simulink model "SonModel"  (R2025b)
settings: Solver=ode4  StartTime=0.0  StopTime=30  FixedStep=0.005  RelTol=1e-3
values from neighbouring files (symbols this model uses):
  CA_alpha_rad_vec = [0 2 4 5 6 7 8 9 10 11 12 13 14 15]*pi/180    [CA_RASAero_2DLUT_Gokturk_1stageVson.m]
  CA_Mach_vec = [      0.01 0.02 0.03 0.04 0.05 0.06 0.07 0.08 0.09 0.1 0.11 0.12      0.13 0.14 0.15 0.16 0.17 0.18 0.19 0.2 0.21 0.22 0.23 0.24      0.25 0.26 0.27 0.28 0.29 0.3 0.31 0.32 0.33 0.34 0.35 0.36      0.37 0.38 0.39 0.4 0.41 0.42 0.43 0.44 0.45 0.46 0.47 0.48      0.49 0.5 0.51 0.52 0.53 0.54 0.55 0.56 0.57 0.58 0.59 0.6      0.61 0.62 0.63 0.64 0.65 0.66 0.67 0.68 0.69 0.7 0.71 0.72      0.73 0.74  ...(+14344 chars)    [CA_RASAero_2DLUT_Gokturk_1stageVson.m]
  CA_table = [ ... (first row only)    [CA_RASAero_2DLUT_Gokturk_1stageVson.m]
  CN_alpha_rad_vec = [0 2 4 5 6 7 8 9 10 11 12 13 14 15]*pi/180    [CN_RASAero_2DLUT_Gokturk_1stageVson.m]
  CN_Mach_vec = [      0.01 0.02 0.03 0.04 0.05 0.06 0.07 0.08 0.09 0.1 0.11 0.12      0.13 0.14 0.15 0.16 0.17 0.18 0.19 0.2 0.21 0.22 0.23 0.24      0.25 0.26 0.27 0.28 0.29 0.3 0.31 0.32 0.33 0.34 0.35 0.36      0.37 0.38 0.39 0.4 0.41 0.42 0.43 0.44 0.45 0.46 0.47 0.48      0.49 0.5 0.51 0.52 0.53 0.54 0.55 0.56 0.57 0.58 0.59 0.6      0.61 0.62 0.63 0.64 0.65 0.66 0.67 0.68 0.69 0.7 0.71 0.72      0.73 0.74  ...(+14344 chars)    [CN_RASAero_2DLUT_Gokturk_1stageVson.m]
  CN_table = [ ... (first row only)    [CN_RASAero_2DLUT_Gokturk_1stageVson.m]
  CP_alpha_rad_vec = [0 2 4 5 6 7 8 9 10 11 12 13 14 15]*pi/180    [CP_RASAero_2DLUT_Gokturk_1stageVson.m]
  CP_Mach_vec = [      0.01 0.02 0.03 0.04 0.05 0.06 0.07 0.08 0.09 0.1 0.11 0.12      0.13 0.14 0.15 0.16 0.17 0.18 0.19 0.2 0.21 0.22 0.23 0.24      0.25 0.26 0.27 0.28 0.29 0.3 0.31 0.32 0.33 0.34 0.35 0.36      0.37 0.38 0.39 0.4 0.41 0.42 0.43 0.44 0.45 0.46 0.47 0.48      0.49 0.5 0.51 0.52 0.53 0.54 0.55 0.56 0.57 0.58 0.59 0.6      0.61 0.62 0.63 0.64 0.65 0.66 0.67 0.68 0.69 0.7 0.71 0.72      0.73 0.74  ...(+14344 chars)    [CP_RASAero_2DLUT_Gokturk_1stageVson.m]
  CP_table = [ ... (first row only)    [CP_RASAero_2DLUT_Gokturk_1stageVson.m]
undefined symbols (not defined in the file or in its folder): Cg, dCA_table, dCm_table, dCN_table, delta_max, g, I_total, KTS_alpha_rad_vec, KTS_delta_rad_vec, KTS_Mach_vec, m_propellant, m_rocket, servo_rate, servo_tau, Sref, thrust, time, time2
libraries: simulink_extras x7, simulink x3, aerolibobsolete x1, slpidlib x1, aerolibatmos2 x1
(part 1 of 2)
settings Model: Creator=aliki  LastModifiedBy=aliki

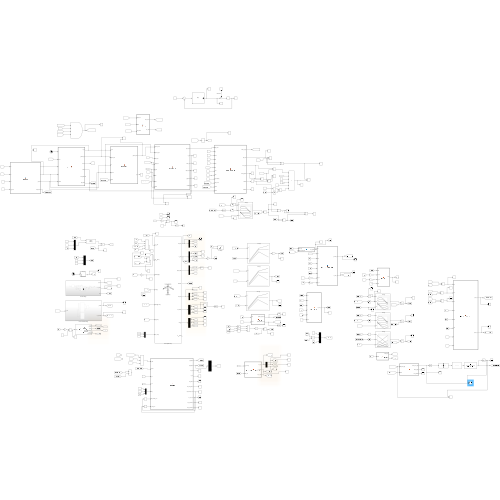
[thumbnail: Simulink's stored preview of the top-level diagram]
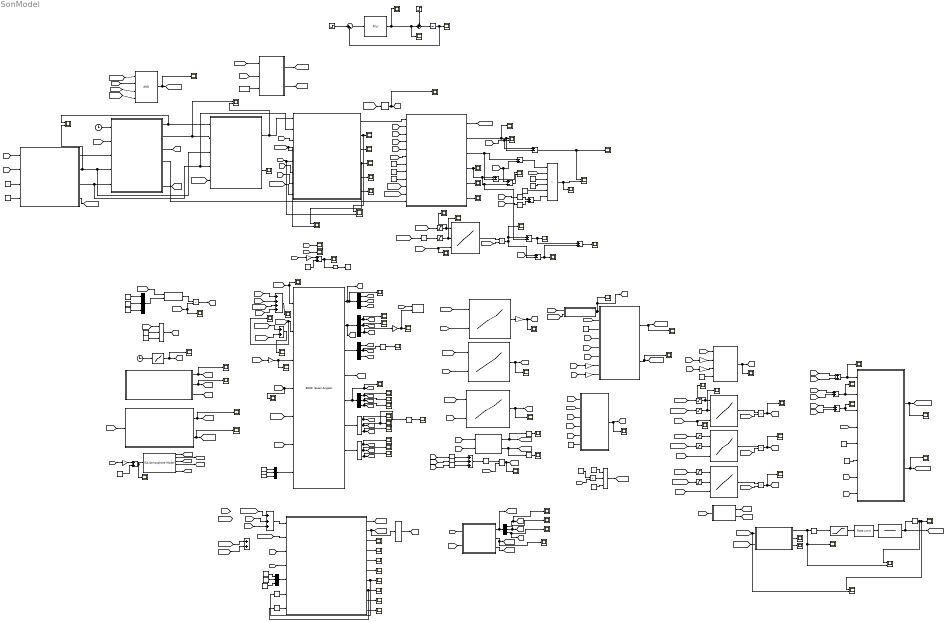
== system SonModel ==
  1-D Lookup Table : Lookup_n-D  NumberOfTableDimensions=1  BreakpointsForDimension1=time2  Table=Cg  InternalRulePriority=Speed  RndMeth=Simplest
  2-D Lookup Table : Lookup_n-D  BreakpointsForDimension1=CA_alpha_rad_vec  BreakpointsForDimension2=CA_Mach_vec  Table=CA_table  ExtrapMethod=Clip  InternalRulePriority=Speed  RndMeth=Simplest
      settings: InputPortMap=u0,u1
  2-D Lookup Table1 : Lookup_n-D  BreakpointsForDimension1=CN_alpha_rad_vec  BreakpointsForDimension2=CN_Mach_vec  Table=CN_table  InternalRulePriority=Speed  RndMeth=Simplest
      settings: InputPortMap=u0,u1
  2-D Lookup Table2 : Lookup_n-D  BreakpointsForDimension1=CP_alpha_rad_vec  BreakpointsForDimension2=CP_Mach_vec  Table=CP_table  InternalRulePriority=Speed  RndMeth=Simplest
      settings: InputPortMap=u0,u1
  6DOF (Quaternion) : aerolibobsolete/6DOF (Euler Angles)  units=Metric (MKS)  mtype=Custom Variable  rep=Quaternion  xme_0=[0 0 0]  Vm_0=[0 0 0]  eul_0=[0 45*pi/180 0]  pm_0=[0 0 0]  mass_0=17.958  mass_e=15.467  mass_f=17.958  inertia=eye(3)  inertia_e=[0.03 0 0; 0 2.263 0; 0 0 2.263]  inertia_f=[0.033 0 0; 0 2.95 0; 0 0 2.95]  k_quat=1.0  vre_flag=on  abi_flag=off  aMode=0  xme_statename=''  Vm_statename=''  eul_statename=''  quat_statename=''  pm_statename=''  mass_statename=''
  AND : Logic  Inputs=4  IconShape=distinctive  AllPortsSameDT=off  OutDataTypeStr=boolean
  Add : Sum  Inputs=++++
  Add{1..2,4,7..9,11..12,17} (9 alike) : Sum
  Add10 : Sum  Inputs=-+
  Add{6,13..16} (5 alike) : Sum  Inputs=+-
  Add3 : Sum  Inputs=+++
  Add5 : Sum  Inputs=+++
  Clock : Clock
  Clock1 : Clock
  Compare To Zero2 : simulink/Logic and Bit Operations/Compare To Zero  relop=<=  OutDataTypeStr=boolean
  Constant{,1..5,7..8,12..14,16,20..21,24} (15 alike) : Constant  Value=0
  Constant10 : Constant
  Constant{6,11,19,23,27} (5 alike) : Constant  Value=Sref
  Constant15 : Constant  Value=9.81
  Constant{17..18,22,26} (4 alike) : Constant  Value=0.122
  Constant25 : Constant  Value=dCm_table
  Constant28 : Constant  Value=0.5
  Constant9 : Constant  Value=970
  Degrees to Radians : simulink_extras/Transformations/Degrees to Radians
  Degrees to Radians1 : simulink_extras/Transformations/Degrees to Radians
  Demux{,1..7} (8 alike) : Demux  Outputs=3
  Discrete PID Controller : slpidlib/PID Controller  Controller=PI  Form=Parallel  TimeDomain=Discrete-time  UseExternalTs=off  SampleTime=0.01  IntegratorMethod=Forward Euler  FilterMethod=Forward Euler  ControllerParametersSource=internal  P=1  I=1  UseKiTs=off  D=0  UseExternalDerivativeSource=off  N=100  UseFilter=on  TunerSelectOption=Transfer Function Based (PID Tuner App)  InitialConditionSource=internal  InitialConditionForIntegrator=0  InitialConditionForFilter=0  DifferentiatorICPrevScaledInput=0  ExternalReset=none  TrackingMode=off  Kt=1  LimitOutput=on  SatLimitsSource=internal  UpperSaturationLimit=0.5  LowerSaturationLimit=-0.5  LinearizeAsGain=off  AntiWindupMode=back-calculation  Kb=1  LimitIntegrator=off  UpperIntegratorSaturationLimit=inf  LowerIntegratorSaturationLimit=-inf  POutMin=[]  POutMax=[]  IOutMin=[]  IOutMax=[]  DOutMin=[]  DOutMax=[]  NOutMin=[]  NOutMax=[]  SumOutMin=[]  SumOutMax=[]  SaturationOutMin=[]  SaturationOutMax=[]  PParamMin=[]  PParamMax=[]  IParamMin=[]  IParamMax=[]  DParamMin=[]  DParamMax=[]  NParamMin=[]  NParamMax=[]  KbParamMin=[]  KbParamMax=[]  KtParamMin=[]  KtParamMax=[]  KbOutMin=[]  KbOutMax=[]  KtOutMin=[]  KtOutMax=[]  IntegratorOutMin=[]  IntegratorOutMax=[]  FilterOutMin=[]  FilterOutMax=[]  SumI1OutMin=[]  SumI1OutMax=[]  SumI2OutMin=[]  SumI2OutMax=[]  SumI3OutMin=[]  SumI3OutMax=[]  SumI4OutMin=[]  SumI4OutMax=[]  SumDOutMin=[]  SumDOutMax=[]  DifferentiatorOutMin=[]  DifferentiatorOutMax=[]  FilterDiffOutCoefMin=[]  FilterDiffOutCoefMax=[]  ReciprocalOutMin=[]  ReciprocalOutMax=[]  SumDenOutMin=[]  SumDenOutMax=[]  SumNumOutMin=[]  SumNumOutMax=[]  DivideOutMin=[]  DivideOutMax=[]  UdiffTsProdOutMin=[]  UdiffTsProdOutMax=[]  NTsProdOutMin=[]  NTsProdOutMax=[]  UintegralTsProdOutMin=[]  UintegralTsProdOutMax=[]  UngainTsProdOutMin=[]  UngainTsProdOutMax=[]  ClampingZeroOutDataTypeStr=Inherit: Inherit via back propagation  ClampingZeroOutMin=[]  ClampingZeroOutMax=[]  FilterDenConstantOutDataTypeStr=Inherit: Inherit via back propagation  FilterDenConstantOutMin=[]  FilterDenConstantOutMax=[]  PCopyOutDataTypeStr=Inherit: Inherit via back propagation  PCopyOutMin=[]  PCopyOutMax=[]  NCopyOutDataTypeStr=Inherit: Inherit via back propagation  NCopyOutMin=[]  NCopyOutMax=[]  IntegratorContinuousStateAttributes=''  IntegratorStateMustResolveToSignalObject=off  IntegratorRTWStateStorageClass=Auto  FilterContinuousStateAttributes=''  FilterStateMustResolveToSignalObject=off  FilterRTWStateStorageClass=Auto  ParallelPVariant=InternalParameters  IdealPVariant=Disabled  IVariant=InternalParameters  DVariant=Disabled  IntegratorVariant=Discrete  SatVariant=Enabled  AWVariant=BackCalculation  PCopyVariant=Disabled  TRVariant=Disabled  FdbkBlocksVariant=Forward  IdealPFdbkVariant=Disabled  SatFdbkVariant=Disabled  DerivativeFilterVariant=Disabled  NVariant=Disabled  NCopyVariant=Disabled_SignalSpec  FilterICVariant=Disabled  IntegratorICVariant=InternalICs  ExternalResetVariant=Disabled  TRSumVariant=Passthrough  SumFdbkVariant=Disabled  SumVariant=Sum_PI  TsampFilterVariant=InternalTs  TsampNgainVariant=Passthrough  TsampIntegralVariant=Disabled_SignalSpec  ExternalSaturationOutDataTypeStr=Inherit: Same as second input  DerivativeSourceVariant=Disabled  PreIntVariant=InternalPreInt
      settings: LibrarySourceBlock=simulink/Discrete/Discrete PID Controller
  Divide : Product  Inputs=*/
  Gain{,1..3} (4 alike) : Gain  Gain=-1
  Gain{5..6,10..11} (4 alike) : Gain  Gain=0.01
  Gain4 : Gain  Gain=2.54
  ISA Atmosphere Model : aerolibatmos2/ISA Atmosphere Model  useExtended=off  action=Warning  custom=off  viscosityOut=on  g=9.80665  gamma=1.4  R=287.0531  L=0.0065  h_trop=11000  h_strat=20000  rho0=1.225  P0=101325  T0=288.15  h0=0  S=110.4  Tref=273.15  muref=1.716e-5
  Inertia of Moment Bloğu : Subsystem
  Integrator : Integrator
  MATLAB Function : MATLAB Function  TreatAsAtomicUnit=on
  MATLAB Function1 : MATLAB Function  TreatAsAtomicUnit=on
  MATLAB Function10 : MATLAB Function  TreatAsAtomicUnit=on
  MATLAB Function11 : MATLAB Function  TreatAsAtomicUnit=on
  MATLAB Function12 : MATLAB Function  TreatAsAtomicUnit=on
  MATLAB Function19 : MATLAB Function  TreatAsAtomicUnit=on
  MATLAB Function2 : MATLAB Function  TreatAsAtomicUnit=on
  MATLAB Function20 : MATLAB Function  TreatAsAtomicUnit=on
  MATLAB Function21 : MATLAB Function  TreatAsAtomicUnit=on
  MATLAB Function3 : MATLAB Function  TreatAsAtomicUnit=on
  MATLAB Function4 : MATLAB Function  TreatAsAtomicUnit=on
  MATLAB Function5 : MATLAB Function  TreatAsAtomicUnit=on
  MATLAB Function6 : MATLAB Function  TreatAsAtomicUnit=on
  MATLAB Function7 : MATLAB Function  TreatAsAtomicUnit=on
  MATLAB Function8 : MATLAB Function  TreatAsAtomicUnit=on
  MATLAB Function9 : MATLAB Function  TreatAsAtomicUnit=on
  Matrix Multiply : Product  Multiplication=Matrix(*)
  Memory : Memory
  Memory1 : Memory
  Mux{,1..3,7} (5 alike) : Mux  Inputs=3
  Product{,1..4,6} (6 alike) : Product
  Product5 : Product  Inputs=6
  Radians to Degrees{,2..4,8} (5 alike) : simulink_extras/Transformations/Radians to Degrees
  Rate Limiter : RateLimiter  RisingSlewLimit=servo_rate  FallingSlewLimit=-servo_rate  SampleTimeMode=inherited
  Saturation{1,3,5,8} (4 alike) : Saturate  UpperLimit=10*pi/180  LowerLimit=-10*pi/180
  Saturation{2,4,6,9} (4 alike) : Saturate  UpperLimit=15*pi/180  LowerLimit=-15*pi/180
  Saturation7 : Saturate  UpperLimit=delta_max  LowerLimit=-delta_max
  Scope{,1..52,55..75,81..88,90..98,100..102} (94 alike) : Scope
      Scope settings: ActiveDisplayYMinimum=-0.1747972451799486  ActiveDisplayYMaximum=1.5731752066195377  DataLoggingVariableName=ScopeData8
      Scope1 settings: ActiveDisplayYMinimum=-1  ActiveDisplayYMaximum=1  DataLoggingVariableName=ScopeData4
      Scope10 settings: ActiveDisplayYMinimum=-0.93845  ActiveDisplayYMaximum=0.10427  DataLoggingVariableName=ScopeData7
      Scope100 settings: ActiveDisplayYMinimum=-1  ActiveDisplayYMaximum=1  DataLoggingVariableName=ScopeData102
      Scope101 settings: ActiveDisplayYMinimum=-1  ActiveDisplayYMaximum=1  DataLoggingVariableName=ScopeData103
      Scope102 settings: ActiveDisplayYMinimum=-1  ActiveDisplayYMaximum=1  DataLoggingVariableName=ScopeData104
      Scope11 settings: ActiveDisplayYMinimum=-126.41054  ActiveDisplayYMaximum=1126.59022  DataLoggingVariableName=ScopeData9
      Scope12 settings: ActiveDisplayYMinimum=0.29833879829396825  ActiveDisplayYMaximum=0.424810785091039  DataLoggingVariableName=ScopeData14
      Scope13 settings: ActiveDisplayYMinimum=-243.41633521256097  ActiveDisplayYMaximum=178.21487911967125  DataLoggingVariableName=ScopeData15
      Scope14 settings: ActiveDisplayYMinimum=19.81436  ActiveDisplayYMaximum=24.47174  DataLoggingVariableName=ScopeData12
      Scope15 settings: ActiveDisplayYMinimum=-1  ActiveDisplayYMaximum=1  DataLoggingVariableName=ScopeData16
      Scope16 settings: ActiveDisplayYMinimum=-1  ActiveDisplayYMaximum=1  DataLoggingVariableName=ScopeData17
      Scope17 settings: ActiveDisplayYMinimum=-1  ActiveDisplayYMaximum=1  DataLoggingVariableName=ScopeData18
      Scope18 settings: ActiveDisplayYMinimum=-59.330334315595763  ActiveDisplayYMaximum=56.592259368399539  DataLoggingVariableName=ScopeData19
      Scope19 settings: ActiveDisplayYMinimum=-1  ActiveDisplayYMaximum=1  DataLoggingVariableName=ScopeData20
      Scope2 settings: ActiveDisplayYMinimum=-1.4090022913253195  ActiveDisplayYMaximum=4.3733572920446138  DataLoggingVariableName=ScopeData5
      Scope20 settings: ActiveDisplayYMinimum=-6.6094473257479365  ActiveDisplayYMaximum=42.313418546311887  DataLoggingVariableName=ScopeData21
      Scope21 settings: ActiveDisplayYMinimum=-0.94288603084583844  ActiveDisplayYMaximum=16.06391617430295  DataLoggingVariableName=ScopeData22
      Scope22 settings: ActiveDisplayYMinimum=-1  ActiveDisplayYMaximum=1  DataLoggingVariableName=ScopeData23
      Scope23 settings: ActiveDisplayYMinimum=-1382.8567732883002  ActiveDisplayYMaximum=1861.3819910244279  DataLoggingVariableName=ScopeData24
      Scope24 settings: ActiveDisplayYMinimum=-0.53683574879227036  ActiveDisplayYMaximum=2.1352657004830919  DataLoggingVariableName=ScopeData25
      Scope25 settings: DataLoggingVariableName=ScopeData26
      Scope26 settings: DataLoggingVariableName=ScopeData27
      Scope27 settings: ActiveDisplayYMinimum=-145.18591664950824  ActiveDisplayYMaximum=126.57706185052312  DataLoggingVariableName=ScopeData28
      Scope28 settings: DataLoggingVariableName=ScopeData29
      Scope29 settings: ActiveDisplayYMinimum=-1.5812738929248127  ActiveDisplayYMaximum=31.007302795539765  DataLoggingVariableName=ScopeData30
      Scope3 settings: ActiveDisplayYMinimum=-3.7763488939592223E-14  ActiveDisplayYMaximum=3.3987140045633005E-13  DataLoggingVariableName=ScopeData6
      Scope30 settings: DataLoggingVariableName=ScopeData31
      Scope31 settings: ActiveDisplayYMinimum=-215.38302091224409  ActiveDisplayYMaximum=1333.9110998732485  DataLoggingVariableName=ScopeData32
      Scope32 settings: ActiveDisplayYMinimum=-60.961188742354921  ActiveDisplayYMaximum=292.29780064349052  DataLoggingVariableName=ScopeData33
      Scope33 settings: ActiveDisplayYMinimum=-1  ActiveDisplayYMaximum=1  DataLoggingVariableName=ScopeData34
      Scope34 settings: ActiveDisplayYMinimum=-10.213165082817136  ActiveDisplayYMaximum=5.7362215763413911  DataLoggingVariableName=ScopeData35
      Scope35 settings: ActiveDisplayYMinimum=13.967875  ActiveDisplayYMaximum=16.859125  DataLoggingVariableName=ScopeData41
      Scope36 settings: ActiveDisplayYMinimum=-0.075411714686402162  ActiveDisplayYMaximum=0.67870543217761958  DataLoggingVariableName=ScopeData42
      Scope37 settings: ActiveDisplayYMinimum=-1  ActiveDisplayYMaximum=1  DataLoggingVariableName=ScopeData43
      Scope38 settings: ActiveDisplayYMinimum=-1  ActiveDisplayYMaximum=1  DataLoggingVariableName=ScopeData36
      Scope39 settings: ActiveDisplayYMinimum=-0.39524232949825433  ActiveDisplayYMaximum=0.24892427629796476  DataLoggingVariableName=ScopeData37
      Scope4 settings: DataLoggingVariableName=ScopeData10
      Scope40 settings: ActiveDisplayYMinimum=-1.0507246376811596  ActiveDisplayYMaximum=1.0492753623188404  DataLoggingVariableName=ScopeData38
      Scope41 settings: ActiveDisplayYMinimum=-234.94308849784304  ActiveDisplayYMaximum=263.75034579370686  DataLoggingVariableName=ScopeData39
      Scope42 settings: ActiveDisplayYMinimum=-34.896271339282123  ActiveDisplayYMaximum=227.8841911010434  DataLoggingVariableName=ScopeData40
      Scope43 settings: ActiveDisplayYMinimum=-2.2084701107262994  ActiveDisplayYMaximum=0.73352279981538893  DataLoggingVariableName=ScopeData44
      Scope44 settings: ActiveDisplayYMinimum=-1  ActiveDisplayYMaximum=1  DataLoggingVariableName=ScopeData45
      Scope45 settings: ActiveDisplayYMinimum=-1  ActiveDisplayYMaximum=1  DataLoggingVariableName=ScopeData46
      Scope46 settings: ActiveDisplayYMinimum=-0.29696656165852287  ActiveDisplayYMaximum=0.23802552760067755  DataLoggingVariableName=ScopeData47
      Scope47 settings: ActiveDisplayYMinimum=-1  ActiveDisplayYMaximum=1  DataLoggingVariableName=ScopeData48
      Scope48 settings: ActiveDisplayYMinimum=-1  ActiveDisplayYMaximum=1  DataLoggingVariableName=ScopeData49
      Scope49 settings: ActiveDisplayYMinimum=-1  ActiveDisplayYMaximum=1  DataLoggingVariableName=ScopeData50
      Scope5 settings: ActiveDisplayYMinimum=-253.26660929354159  ActiveDisplayYMaximum=3684.2383287363355  DataLoggingVariableName=ScopeData11
      Scope50 settings: ActiveDisplayYMinimum=-8.4467484261868346  ActiveDisplayYMaximum=8.27792222569828  DataLoggingVariableName=ScopeData51
      Scope51 settings: ActiveDisplayYMinimum=-102.02541516324928  ActiveDisplayYMaximum=52.893082782127507  DataLoggingVariableName=ScopeData52
      Scope52 settings: ActiveDisplayYMinimum=-5.4877093696950805  ActiveDisplayYMaximum=6.0180574574424348  DataLoggingVariableName=ScopeData54
      Scope55 settings: ActiveDisplayYMinimum=-5.8365353519896939  ActiveDisplayYMaximum=5.8301335116870519  DataLoggingVariableName=ScopeData57
      Scope56 settings: DataLoggingVariableName=ScopeData58
      Scope57 settings: ActiveDisplayYMinimum=0.1417978480190214  ActiveDisplayYMaximum=0.72381936782880774  DataLoggingVariableName=ScopeData59
      Scope58 settings: ActiveDisplayYMinimum=-1  ActiveDisplayYMaximum=1  DataLoggingVariableName=ScopeData60
      Scope59 settings: ActiveDisplayYMinimum=-14.122932548575566  ActiveDisplayYMaximum=11.11801932115314  DataLoggingVariableName=ScopeData61
      Scope6 settings: ActiveDisplayYMinimum=-88.915261777404467  ActiveDisplayYMaximum=795.20104066911313  DataLoggingVariableName=ScopeData13
      Scope60 settings: ActiveDisplayYMinimum=-1.47242975885713  ActiveDisplayYMaximum=0.80090322626159427  DataLoggingVariableName=ScopeData62
      Scope61 settings: ActiveDisplayYMinimum=-21.480582324133742  ActiveDisplayYMaximum=26.46311961535914  DataLoggingVariableName=ScopeData63
      Scope62 settings: ActiveDisplayYMinimum=-1  ActiveDisplayYMaximum=1  DataLoggingVariableName=ScopeData64
      Scope63 settings: ActiveDisplayYMinimum=-5.4515031776112985E-14  ActiveDisplayYMaximum=5.5734968223887031E-14  DataLoggingVariableName=ScopeData65
      Scope64 settings: ActiveDisplayYMinimum=83.8517506647575  ActiveDisplayYMaximum=104.85175066475749  DataLoggingVariableName=ScopeData66
      Scope65 settings: ActiveDisplayYMinimum=-6.6505514678807653  ActiveDisplayYMaximum=6.7448325642623788  DataLoggingVariableName=ScopeData67
      Scope66 settings: DataLoggingVariableName=ScopeData68
      Scope67 settings: DataLoggingVariableName=ScopeData69
      Scope68 settings: DataLoggingVariableName=ScopeData70
      Scope69 settings: DataLoggingVariableName=ScopeData71
      Scope7 settings: ActiveDisplayYMinimum=-378.89044493527791  ActiveDisplayYMaximum=3410.0140044175018
      Scope70 settings: DataLoggingVariableName=ScopeData72
      Scope71 settings: DataLoggingVariableName=ScopeData73
      Scope72 settings: DataLoggingVariableName=ScopeData74
      Scope73 settings: ActiveDisplayYMinimum=-1  ActiveDisplayYMaximum=1  DataLoggingVariableName=ScopeData75
      Scope74 settings: DataLoggingVariableName=ScopeData76
      Scope75 settings: DataLoggingVariableName=ScopeData77
      Scope8 settings: ActiveDisplayYMinimum=-1  ActiveDisplayYMaximum=1  DataLoggingVariableName=ScopeData3
      Scope81 settings: ActiveDisplayYMinimum=-1  ActiveDisplayYMaximum=1  DataLoggingVariableName=ScopeData83
      Scope82 settings: ActiveDisplayYMinimum=-0.33071620318847983  ActiveDisplayYMaximum=0.399993974324673  DataLoggingVariableName=ScopeData84
      Scope83 settings: ActiveDisplayYMinimum=3.066715815282711  ActiveDisplayYMaximum=4.0559204649685876  DataLoggingVariableName=ScopeData85
      Scope84 settings: ActiveDisplayYMinimum=-1  ActiveDisplayYMaximum=1  DataLoggingVariableName=ScopeData86
      Scope85 settings: ActiveDisplayYMinimum=-1  ActiveDisplayYMaximum=1  DataLoggingVariableName=ScopeData87
      Scope86 settings: ActiveDisplayYMinimum=-0.39524232949825433  ActiveDisplayYMaximum=0.24892427629796476  DataLoggingVariableName=ScopeData88
      Scope87 settings: ActiveDisplayYMinimum=-1.0507246376811596  ActiveDisplayYMaximum=1.0492753623188404  DataLoggingVariableName=ScopeData89
      Scope88 settings: ActiveDisplayYMinimum=-4.3465798396882604  ActiveDisplayYMaximum=7.4540792632747968  DataLoggingVariableName=ScopeData90
      Scope9 settings: ActiveDisplayYMinimum=-88.533632277198407  ActiveDisplayYMaximum=806.80269049478579  DataLoggingVariableName=ScopeData53
      Scope90 settings: DataLoggingVariableName=ScopeData92
      Scope91 settings: ActiveDisplayYMinimum=-1.0788840221514682  ActiveDisplayYMaximum=1.0773897507630206  DataLoggingVariableName=ScopeData93
      Scope92 settings: DataLoggingVariableName=ScopeData94
      Scope93 settings: ActiveDisplayYMinimum=0.1417978480190214  ActiveDisplayYMaximum=0.72381936782880774  DataLoggingVariableName=ScopeData95
      Scope94 settings: ActiveDisplayYMinimum=-6.8859273941263011E-5  ActiveDisplayYMaximum=3.6121632887214927E-5  DataLoggingVariableName=ScopeData96
      Scope95 settings: ActiveDisplayYMinimum=-0.077719610652531537  ActiveDisplayYMaximum=0.020454605179062134  DataLoggingVariableName=ScopeData97
      Scope96 settings: ActiveDisplayYMinimum=-0.036073362961241508  ActiveDisplayYMaximum=0.018695728425076431  DataLoggingVariableName=ScopeData98
      Scope97 settings: DataLoggingVariableName=ScopeData99
      Scope98 settings: DataLoggingVariableName=ScopeData100
  Scope{53..54,76..80,89,99} (9 alike) : Scope  NumInputPorts=2
      Scope53 settings: ActiveDisplayYMinimum=-0.9647475155961196  ActiveDisplayYMaximum=0.1433853526765958  DataLoggingVariableName=ScopeData55
      Scope54 settings: ActiveDisplayYMinimum=-0.13985800272274002  ActiveDisplayYMaximum=0.33625240802956446  DataLoggingVariableName=ScopeData56
      Scope76 settings: ActiveDisplayYMinimum=-116.96927485132606  ActiveDisplayYMaximum=808.85109522524442  DataLoggingVariableName=ScopeData78
      Scope77 settings: ActiveDisplayYMinimum=-1.0463543969685811  ActiveDisplayYMaximum=0.8902654705070111  DataLoggingVariableName=ScopeData79
      Scope78 settings: ActiveDisplayYMinimum=-0.11516989219555035  ActiveDisplayYMaximum=0.022921378974532808  DataLoggingVariableName=ScopeData80
      Scope79 settings: ActiveDisplayYMinimum=-0.16793116661559071  ActiveDisplayYMaximum=0.061329013063235682  DataLoggingVariableName=ScopeData81
      Scope80 settings: ActiveDisplayYMinimum=-5.6977882125045722  ActiveDisplayYMaximum=5.2077545596519705  DataLoggingVariableName=ScopeData82
      Scope89 settings: ActiveDisplayYMinimum=-0.015084051232345921  ActiveDisplayYMaximum=0.014890107412311292  DataLoggingVariableName=ScopeData91
      Scope99 settings: ActiveDisplayYMinimum=-6.6004039221544462  ActiveDisplayYMaximum=4.0784881107001141  DataLoggingVariableName=ScopeData101
  Selector : Selector  NumberOfDimensions=2  InputPortWidth=3  IndexOptions=Index vector (dialog),Index vector (dialog)  Indices=2,2  OutputSizes=1,1
  Sqrt : Sqrt
  Square{,1..4} (5 alike) : Math  Operator=square
  Step : Step  Time=0  SampleTime=0
  Step1 : Step  Time=5  After=0.2  SampleTime=0
  Stop Simulation : Stop
  Sum : Sum  Inputs=|+-
  Sum1 : Sum  Inputs=++|
  Transfer Fcn : TransferFcn  Denominator=[servo_tau 1]
  XY Graph : Record  NumPorts=2.0  FileSettingsInternal="{\"entries\":[{\"content\":{\"excelSettings\":{\"content\":{},\"type\":\"Streamout.ExcelSettings\"},\"parquetSettings\":{\"content\":{},\"type\":\"Streamout.ParquetSettings\"}},\"type\":\"Streamout.FileSettingStorage\",\"uuid\":\"\"}],\"packageUris\":[\"http:\\/\\/schema.mathworks.com\\/mf0\\/streamout_blocks\\/R2020a\"],\"version\":\"1.0\"}"  FrameSettings=[0, 0]  Layout=[1 1]  SignalsInternal="{\"entries\":[{\"content\":{\"signals\":[{\"content\":{\"blockPath\":[],\"dimensions\":[1],\"domain\":\"\",\"lineColor\":\"#a2142f\",\"lineWidth\":2,\"port\":1,\"sid\":[\"\"],\"signalID\":1,\"signalName\":\"From90\"},\"type\":\"RecordBlkView.Signal\",\"uuid\":\"\"},{\"content\":{\"blockPath\":[],\"dimensions\":[1],\"domain\":\"\",\"lineColor\":\"#139fff\",\"lineWidth\":2,\"port\":2,\"sid\":[\"\"],\"signalID\":2,\"signalName\":\"Gain3\"},\"type\":\"RecordBlkView.Signal\",\"uuid\":\"\"}]},\"type\":\"RecordBlkView.InputSignals\",\"uuid\":\"\"}],\"packageUris\":[\"http:\\/\\/schema.mathworks.com\\/mf0\\/streamout_blocks\\/R2020a\"],\"version\":\"1.0\"}"  VisualizationBindings="{\"xyplotplugin\":{\"info\":[{\"series\":[],\"subplotID\":1}]}}"  CompatibilityTag=XY
  kq : Constant  Value=-0.3
  n-D Lookup Table : Lookup_n-D  NumberOfTableDimensions=3  BreakpointsForDimension1=KTS_alpha_rad_vec  BreakpointsForDimension2=KTS_delta_rad_vec  BreakpointsForDimension3=KTS_Mach_vec  Table=dCm_table  InternalRulePriority=Speed  RndMeth=Simplest
      settings: InputPortMap=u0,u1,u2
  n-D Lookup Table1 : Lookup_n-D  NumberOfTableDimensions=3  BreakpointsForDimension1=KTS_alpha_rad_vec  BreakpointsForDimension2=KTS_delta_rad_vec  BreakpointsForDimension3=KTS_Mach_vec  Table=dCN_table  InternalRulePriority=Speed  RndMeth=Simplest
      settings: InputPortMap=u0,u1,u2
  n-D Lookup Table2 : Lookup_n-D  NumberOfTableDimensions=3  BreakpointsForDimension1=KTS_alpha_rad_vec  BreakpointsForDimension2=KTS_delta_rad_vec  BreakpointsForDimension3=KTS_Mach_vec  Table=dCA_table  InternalRulePriority=Speed  RndMeth=Simplest
      settings: InputPortMap=u0,u1,u2
  n-D Lookup Table3 : Lookup_n-D  NumberOfTableDimensions=3  BreakpointsForDimension1=KTS_alpha_rad_vec  BreakpointsForDimension2=KTS_delta_rad_vec  BreakpointsForDimension3=KTS_Mach_vec  Table=dCm_table  InternalRulePriority=Speed  RndMeth=Simplest
      settings: InputPortMap=u0,u1,u2
  İtki-Kütle Bloğu : Subsystem
  wires:
  [m_dot] -> Inertia of Moment Bloğu/1(m_dot)
  Constant14/1 -> Mux3/2
  [DCMbe] -> Matrix Multiply/1
  ISA Atmosphere Model/3 -> [basinc]
  ISA Atmosphere Model/4 -> [rho]
  Constant9/1 -> Add1/2
  İtki-Kütle Bloğu/2(m_roket) -> Scope4/1, [m_roket]
  Constant8/1 -> Mux2/3
  Clock/1 -> 1-D Lookup Table/1
  [m_roket] -> Product4/2, Scope14/1
  Add1/1 -> ISA Atmosphere Model/1, Scope11/1
  Mux3/1 -> Matrix Multiply/2
  1-D Lookup Table/1 -> Scope17/1, [cg]  "cg"
  Constant13/1 -> Mux3/1
  İtki-Kütle Bloğu/3(itki) -> [itki]
  Matrix Multiply/1 -> Product4/1
  Constant15/1 -> Mux3/3
  Constant7/1 -> Mux2/2
  İtki-Kütle Bloğu/1(m_dot) -> Scope/1, [m_dot]
  ISA Atmosphere Model/2 -> [seshizi]
  Gain1/1 -> Add1/1
  [Z] -> Gain1/1
  Product4/1 -> [Fg]
  [itki] -> Mux2/1
  ISA Atmosphere Model/1 -> [Kelvin]
  ISA Atmosphere Model/6 -> [viskozite]
  Mux2/1 -> [Fitki]
  [Fdrag] -> Add/1
  Constant/1 -> Mux/1
  Demux1/2 -> Scope5/1, [Y]
  Constant1/1 -> Mux/3
  Demux1/3 -> Gain3/1, [Z]
  [m_dot] -> Gain/1
  Demux2/1 -> [Phi]
  Demux2/3 -> [Psi]
  6DOF (Quaternion)/4 -> [DCMbe]
  Demux/2 -> [Vy]
  Gain/1 -> Scope10/1, 6DOF (Quaternion)/3
  Radians to Degrees/1 -> Scope18/1
  Demux4/2 -> Radians to Degrees4/1, Scope39/1, [q]
  6DOF (Quaternion)/2 -> [X_e], Demux1/1
  [Fitki] -> Add/2
  Demux/3 -> [Vz]
  Demux4/3 -> Scope40/1, [r]
  Demux3/3 -> Scope34/1, [w]
  Demux/1 -> [Vx]
  6DOF (Quaternion)/5 -> Demux3/1, Scope42/1, [Vb]
  Demux1/1 -> [X], Scope3/1
  6DOF (Quaternion)/1 -> [V_e], Demux/1, Scope41/1
  Demux2/2 -> Radians to Degrees/1, [Theta]
  6DOF (Quaternion)/3 -> Demux2/1
  Constant2/1 -> Mux/2
  Demux3/1 -> Scope32/1, [u]
  Mux/1 -> 6DOF (Quaternion)/7
  Demux4/1 -> [p], Scope38/1
  6DOF (Quaternion)/6 -> Demux4/1
  Compare To Zero2/1 -> Stop Simulation/1
  [Z] -> Gain2/1
  Add2/1 -> Scope9/1, Compare To Zero2/1
  Gain2/1 -> Add2/1
  Constant10/1 -> Add2/2
  [m_roket] -> 6DOF (Quaternion)/4, Scope35/1
  Inertia of Moment Bloğu/1(I_matrix) -> Scope2/1, [I_matrix]
  [I_matrix] -> 6DOF (Quaternion)/6
  Inertia of Moment Bloğu/2(dI_dt_matrix) -> Scope1/1, [dl_dt_matrix]
  [dl_dt_matrix] -> 6DOF (Quaternion)/5
  Gain3/1 -> XY Graph/2, Scope6/1
  Square/1 -> Add3/1
  Square1/1 -> Add3/2
  Square2/1 -> Add3/3
  Add3/1 -> Sqrt/1
  Sqrt/1 -> Divide/1
  [seshizi] -> Divide/2
  2-D Lookup Table/1 -> Scope12/1, [CA0]
  MATLAB Function1/1(F_aero_b) -> [Fdrag], Scope16/1
  [CA0] -> MATLAB Function1/1(CA)
  [rho] -> MATLAB Function1/2(rho)
  [W_air] -> MATLAB Function1/5(w)
  Constant6/1 -> MATLAB Function1/6(Sref)
  Divide/1 -> Scope36/1, [Mach]
  [Mach] -> 2-D Lookup Table/2
  [Mach] -> 2-D Lookup Table1/2
  2-D Lookup Table1/1 -> Scope19/1, [CN]
  [Mach] -> 2-D Lookup Table2/2
  2-D Lookup Table2/1 -> Gain4/1
  Gain4/1 -> Scope64/1, [Cp]
  Gain5/1 -> MATLAB Function2/8(CP_m)
  [Cp] -> Gain5/1
  [cg] -> Gain6/1
  Gain6/1 -> MATLAB Function2/7(CG_m)
  [u_air] -> MATLAB Function2/4(u)
  [W_air] -> MATLAB Function2/6(w)
  Constant11/1 -> MATLAB Function2/3(Sref)
  [rho] -> MATLAB Function2/2(rho)
  MATLAB Function2/1(F_normal_b) -> [F_normal_CN], Scope13/1
  [q] -> Product/2
  kq/1 -> Product/1
  Product/1 -> Mux1/2
  Constant3/1 -> Mux1/3
  Constant4/1 -> Mux1/1
  Mux1/1 -> [q_damping]
  [M_aero_CN] -> Add4/1
  [q_damping] -> Add4/2
  MATLAB Function2/2(M_aero_b) -> Scope15/1, [M_aero_CN]
  [Fg] -> Add/4
  [F_normal_CN] -> Add/3
  MATLAB Function/1(alpha_signed_rad) -> Radians to Degrees2/1, [AoA_signed]
  Radians to Degrees2/1 -> Scope20/1
  [CN] -> MATLAB Function6/1(CN_mag)
  [AoA_signed] -> MATLAB Function6/2(alpha_signed_rad)
  MATLAB Function6/1(CN_signed) -> [CN0], Scope49/1, MATLAB Function2/1(CN)
  MATLAB Function/2(alpha_RASAero_rad) -> [AoA_rasaero], Radians to Degrees3/1
  Radians to Degrees3/1 -> Scope21/1
  [AoA_rasaero] -> 2-D Lookup Table1/1
  [X_e] -> MATLAB Function7/3(X_e)
  [Vb] -> MATLAB Function7/4(V_b)
  MATLAB Function7/1(F_applied) -> [F_applied]
  MATLAB Function7/2(M_applied) -> Demux6/1, [M_applied]
  MATLAB Function7/3(on_rail) -> Scope22/1
  MATLAB Function7/4(s_rail) -> Scope23/1
  MATLAB Function7/5(rail_phase) -> Scope24/1
  MATLAB Function7/6(rail_clear_pulse) -> Scope25/1
  MATLAB Function7/7(rail_cleared_now) -> Memory/1, Scope26/1
  MATLAB Function7/9(F_rail_reaction) -> Scope27/1
  MATLAB Function7/10(M_rail_reaction) -> Scope28/1
  Mux7/1 -> MATLAB Function7/5(X0_e)
  Constant5/1 -> Mux7/1
  Constant12/1 -> Mux7/2
  Constant16/1 -> Mux7/3
  Memory/1 -> MATLAB Function7/6(rail_cleared_prev)
  Memory1/1 -> MATLAB Function7/7(V_exit_prev)
  MATLAB Function7/8(V_exit_now) -> Scope29/1, Memory1/1
  Demux3/2 -> Scope33/1, [v]
  [AoA_signed] -> Saturation1/1
  Saturation1/1 -> Scope30/1, n-D Lookup Table/1
  Saturation2/1 -> Scope56/1, n-D Lookup Table/2
  Saturation4/1 -> n-D Lookup Table1/2
  Saturation3/1 -> n-D Lookup Table1/1
  [AoA_signed] -> Saturation3/1
  Saturation6/1 -> n-D Lookup Table2/2
  Saturation5/1 -> n-D Lookup Table2/1
  [AoA_signed] -> Saturation5/1
  [MachLut] -> n-D Lookup Table1/3
  [MachLut] -> n-D Lookup Table2/3
  [CN0] -> MATLAB Function8/1(CN0)
  [Cp] -> Gain10/1
  Gain11/1 -> MATLAB Function8/2(CG_m)
  [cg] -> Gain11/1
  Gain10/1 -> MATLAB Function8/3(CP_m)
  Constant17/1 -> MATLAB Function8/4(Lref)
  MATLAB Function8/1(Cm0) -> Scope37/1, [Cm0]
  [Cm0] -> Add7/1
  [DelCm] -> Add7/2
  [CN0] -> Add8/1
  [DelCN] -> Add8/2
  [CA0] -> Add9/1
  [DelCA] -> Add9/2
  [Mach] -> MATLAB Function10/1(Mach)
  MATLAB Function10/1(Mach_LUT) -> [MachLut]
  [MachLut] -> n-D Lookup Table/3, Scope57/1
  MATLAB Function10/2(KTS_active) -> [KTS_active]
  n-D Lookup Table2/1 -> Product1/1
  [KTS_active] -> Product1/2
  Product1/1 -> Scope48/1, [DelCA]
  n-D Lookup Table1/1 -> Product2/1
  [KTS_active] -> Product2/2
  Product2/1 -> Scope47/1, [DelCN]
  n-D Lookup Table/1 -> Product3/1
  [KTS_active] -> Product3/2
  Product3/1 -> Scope46/1, [DelCm]
  Add7/1 -> Scope43/1, MATLAB Function9/1(Cm)
  Add8/1 -> MATLAB Function9/2(CN), Scope44/1
  Add9/1 -> MATLAB Function9/3(CA), Scope45/1
  [AoA_rasaero] -> 2-D Lookup Table/1
  [Deflection_actual] -> Saturation2/1
  [Deflection_actual] -> Saturation4/1
  [Deflection_actual] -> Saturation6/1
  [rho] -> MATLAB Function9/4(rho)
  Constant18/1 -> MATLAB Function9/6(Lref)
  Constant19/1 -> MATLAB Function9/5(Sref)
  [u_air] -> MATLAB Function9/7(u)
  [W_air] -> MATLAB Function9/8(w)
  MATLAB Function9/1(F_aero_b) -> Scope51/1, [F_AERO_DEF]
  MATLAB Function9/2(M_aero_b) -> Scope50/1, [M_AERO_DEF]
  Saturation7/1 -> Rate Limiter/1
  Rate Limiter/1 -> Transfer Fcn/1
  [Fitki] -> Add5/2
  Add5/1 -> MATLAB Function7/1(F_raw)
  [M_aero_CN] -> Add11/1
  [q_damping] -> Add11/2
  [Y] -> Scope8/1
  [X] -> Scope7/1
  [X] -> XY Graph/1
  [F_applied] -> 6DOF (Quaternion)/1, Scope31/1
  [M_applied] -> Scope59/1, 6DOF (Quaternion)/2
  Add/1 -> Scope58/1
  Add4/1 -> Scope60/1
  [Vb] -> MATLAB Function11/1(V_ground_b)
  [DCMbe] -> MATLAB Function11/2(DCM_be)
  Demux5/1 -> Scope66/1, [u_air]
  Demux5/2 -> Scope63/1, [v_air]
  MATLAB Function11/3(V_air_mag) -> [V_air_mag]
  [u_air] -> MATLAB Function1/3(u)
  [u_air] -> MATLAB Function/1(u_rel)
  [W_air] -> MATLAB Function/2(w_rel)
  [u_air] -> Square/1
  [v_air] -> Square1/1
  [W_air] -> Square2/1
  Radians to Degrees4/1 -> Scope61/1
  MATLAB Function11/2(V_wind_b) -> Scope62/1, [V_wind_b]
  MATLAB Function11/1(V_air_b) -> [V_air_b], Demux5/1
  [v_air] -> MATLAB Function2/5(v)
  [v_air] -> MATLAB Function1/4(v)
  [AoA_signed] -> 2-D Lookup Table2/1
  Demux5/3 -> [W_air], Scope65/1
  [F_AERO_DEF] -> Add5/1
  [M_AERO_DEF] -> MATLAB Function7/2(M_raw)
  [V_e] -> MATLAB Function5/2(Ve)
  [X_e] -> MATLAB Function5/1(Xe)
  Constant20/1 -> MATLAB Function5/3(x0)
  Constant21/1 -> MATLAB Function5/4(z_ground)
  Clock1/1 -> MATLAB Function19/1(t)
  [itki] -> MATLAB Function19/2(thrust)
  MATLAB Function5/1(x) -> MATLAB Function19/3(x)
  MATLAB Function5/3(gamma) -> MATLAB Function3/2(gamma_gnd), MATLAB Function20/4(gamma), MATLAB Function19/5(gamma)
  MATLAB Function19/1(h_ref) -> Scope76/1, MATLAB Function20/1(h_ref)
  MATLAB Function19/3(active) -> [active]
  MATLAB Function20/1(gamma_cmd) -> Scope77/2, MATLAB Function3/1(gamma_cmd)
  [Theta] -> MATLAB Function3/3(theta_hat)
  [q] -> Scope78/2, MATLAB Function3/5(q_hat)
  MATLAB Function3/1(qdot_cmd) -> MATLAB Function21/1(qdot_cmd)
  [I_matrix] -> Selector/1
  Selector/1 -> Scope83/1, [Iyy]
  [Cm0] -> MATLAB Function21/3(Cm0)
  [rho] -> MATLAB Function21/6(rho)
  Constant23/1 -> MATLAB Function21/7(Sref)
  [W_air] -> MATLAB Function21/5(wair)
  Constant22/1 -> MATLAB Function21/8(cbar)  "Lref"
  [u_air] -> MATLAB Function21/4(uair)
  Constant24/1 -> MATLAB Function21/9(My_damping)
  [AoA_signed] -> MATLAB Function4/1(alpha_rad)
  [Fg] -> Add5/3
  Constant25/1 -> MATLAB Function4/3(dCm_table)
  [MachLut] -> MATLAB Function4/2(Mach)
  MATLAB Function4/1(dCm_curve) -> [dCm_curve]
  [dCm_curve] -> MATLAB Function21/10(dCm_curve)
  MATLAB Function19/4(blend) -> MATLAB Function21/12(blend)
  [u_air] -> MATLAB Function3/6(uair)
  [W_air] -> MATLAB Function3/7(wair)
  MATLAB Function3/3(theta_ref) -> Scope68/1
  MATLAB Function3/5(e_gamma) -> Scope70/1
  MATLAB Function3/6(enabled) -> Scope71/1
  MATLAB Function20/2(e_h) -> Scope72/1
  [Iyy] -> MATLAB Function21/2(Iyy)
  MATLAB Function21/1(delta_e_deg) -> [defkomut_deg]
  MATLAB Function21/3(dCm_req) -> Add13/2, Add10/1
  MATLAB Function21/5(limited) -> Scope74/1
  MATLAB Function21/6(enabled) -> Scope75/1
  MATLAB Function5/4(valid_motion) -> [valid_motion]
  [valid_motion] -> AND/1
  [active] -> AND/2
  MATLAB Function4/2(lut_valid) -> [lut_valid]
  [lut_valid] -> AND/3
  MATLAB Function19/6(path_valid) -> [path_valid]
  [path_valid] -> AND/4
  AND/1 -> Scope84/1, [active_total]
  [active_total] -> MATLAB Function20/5(active)
  [active_total] -> MATLAB Function3/8(active)
  [active_total] -> MATLAB Function21/11(active)
  MATLAB Function19/2(gamma_ref) -> MATLAB Function20/2(gamma_ref), Scope77/1
  MATLAB Function5/2(h) -> MATLAB Function20/3(h), MATLAB Function19/4(h), Scope76/2
  MATLAB Function3/2(q_ref) -> Scope67/1, Scope78/1
  MATLAB Function3/4(alpha_cmd) -> Scope69/1, Scope79/1
  [AoA_signed] -> MATLAB Function3/4(alpha_hat), Scope79/2
  Degrees to Radians/1 -> Saturation7/1
  Demux6/2 -> [My]
  [My] -> Add6/1, Scope53/2
  MATLAB Function21/2(My_cmd) -> Scope81/1, Add6/2, Scope53/1
  Demux7/1 -> Scope85/1, [p_dot]
  Demux7/3 -> Scope87/1, [r_dot]
  Demux7/2 -> Scope86/1, [q_dot]
  6DOF (Quaternion)/7 -> Demux7/1
  [DelCm] -> Add14/1, Add10/2
  Constant26/1 -> Product5/4  "Lref"
  Constant27/1 -> Product5/3
  Add10/1 -> Product5/1
  [rho] -> Product5/2
  Constant28/1 -> Product5/5
  [u_air] -> Square3/1
  [W_air] -> Square4/1
  Square3/1 -> Add12/1
  Square4/1 -> Add12/2
  Add12/1 -> Product5/6
  Add6/1 -> Scope54/1, Scope82/1
  Product5/1 -> Scope88/1, Scope54/2
  Add13/1 -> Scope89/1
  Add14/1 -> Scope89/2
  Saturation9/1 -> Scope92/1, n-D Lookup Table3/2
  [MachLut] -> n-D Lookup Table3/3, Scope93/1
  n-D Lookup Table3/1 -> Product6/1
  [KTS_active] -> Product6/2
  [AoA_signed] -> Saturation8/1
  Product6/1 -> Add16/2, Add15/1, Scope91/1
  Saturation8/1 -> Scope90/1, n-D Lookup Table3/1
  MATLAB Function21/4(dCm_applied) -> Add15/2, Add14/2, Add13/1, Scope73/1
  Add15/1 -> Add17/1, Scope94/1  "r1"
  [DelCm] -> Add16/1
  Add16/1 -> Add17/2, Scope95/1  "r2"
  Add17/1 -> Scope96/1
  [defkomut_deg] -> Degrees to Radians1/1
  Degrees to Radians1/1 -> Saturation9/1
  [defkomut_deg] -> Scope99/2, MATLAB Function12/1(delta_des_deg)
  MATLAB Function12/2(delta_ff_deg) -> Scope97/1
  MATLAB Function12/3(comp_limited) -> Scope98/1
  Transfer Fcn/1 -> [Deflection_actual], Radians to Degrees8/1
  Radians to Degrees8/1 -> Scope80/1, Scope55/1, Scope99/1
  Sum/1 -> Discrete PID Controller/1
  Step/1 -> Sum/1
  Integrator/1 -> Sum/2, Scope100/1
  Sum1/1 -> Integrator/1
  Step1/1 -> Sum1/1  "Disturbance"
  Discrete PID Controller/1 -> Scope102/1, Sum1/2, Scope101/1
  MATLAB Function12/1(delta_servo_deg) -> Scope80/2, Scope52/1, Degrees to Radians/1
  [active_total] -> MATLAB Function12/2(active)

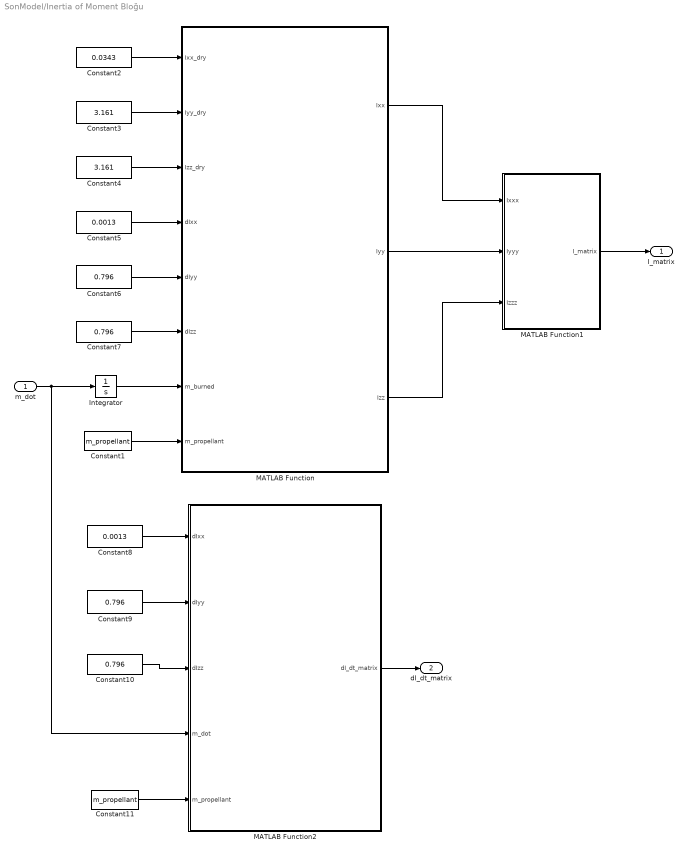
== system SonModel/Inertia of Moment Bloğu ==
  m_dot : Inport
  Constant1 : Constant  Value=m_propellant
  Constant{6..7,9..10} (4 alike) : Constant  Value=0.796
  Constant11 : Constant  Value=m_propellant
  Constant2 : Constant  Value=0.0343
  Constant3 : Constant  Value=3.161
  Constant4 : Constant  Value=3.161
  Constant5 : Constant  Value=0.0013
  Constant8 : Constant  Value=0.0013
  Integrator : Integrator
  MATLAB Function : MATLAB Function  TreatAsAtomicUnit=on
  MATLAB Function1 : MATLAB Function  TreatAsAtomicUnit=on
  MATLAB Function2 : MATLAB Function  TreatAsAtomicUnit=on
  I_matrix : Outport
  dI_dt_matrix : Outport  Port=2
  wires:
  Constant1/1 -> MATLAB Function/8(m_propellant)
  Constant2/1 -> MATLAB Function/1(Ixx_dry)
  Constant3/1 -> MATLAB Function/2(Iyy_dry)
  Constant4/1 -> MATLAB Function/3(Izz_dry)
  Constant5/1 -> MATLAB Function/4(dIxx)
  Constant6/1 -> MATLAB Function/5(dIyy)
  Constant7/1 -> MATLAB Function/6(dIzz)
  MATLAB Function/1(Ixx) -> MATLAB Function1/1(Ixxx)
  MATLAB Function/3(Izz) -> MATLAB Function1/3(Izzz)
  m_dot/1 -> Integrator/1, MATLAB Function2/4(m_dot)
  Integrator/1 -> MATLAB Function/7(m_burned)
  MATLAB Function/2(Iyy) -> MATLAB Function1/2(Iyyy)
  MATLAB Function1/1(I_matrix) -> I_matrix/1
  Constant11/1 -> MATLAB Function2/5(m_propellant)
  MATLAB Function2/1(dI_dt_matrix) -> dI_dt_matrix/1
  Constant8/1 -> MATLAB Function2/1(dIxx)
  Constant9/1 -> MATLAB Function2/2(dIyy)
  Constant10/1 -> MATLAB Function2/3(dIzz)

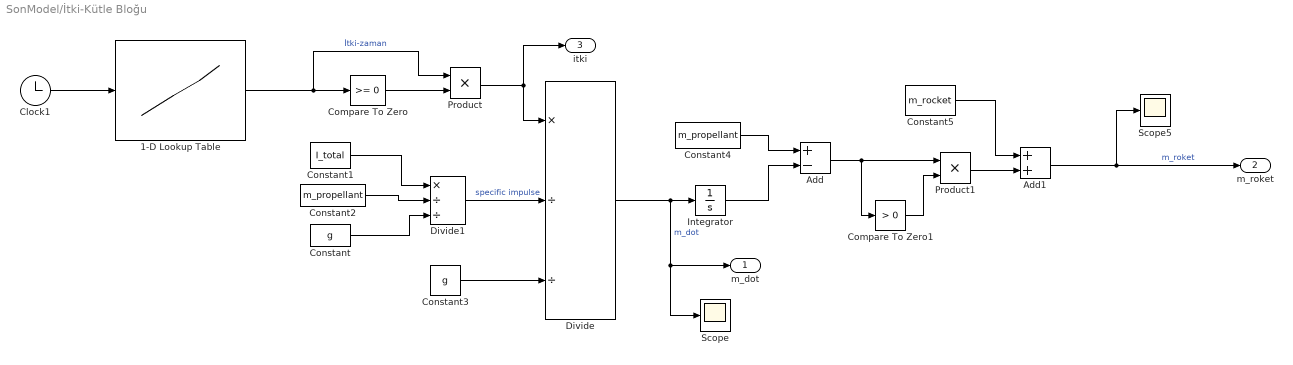
== system SonModel/İtki-Kütle Bloğu ==
  1-D Lookup Table : Lookup_n-D  NumberOfTableDimensions=1  BreakpointsForDimension1=time  Table=thrust  InternalRulePriority=Speed  RndMeth=Simplest
  Add : Sum  Inputs=+-
  Add1 : Sum
  Clock1 : Clock
  Compare To Zero : simulink/Logic and Bit Operations/Compare To Zero  relop=>=  OutDataTypeStr=boolean
  Compare To Zero1 : simulink/Logic and Bit Operations/Compare To Zero  relop=>  OutDataTypeStr=boolean
  Constant : Constant  Value=g  VectorParams1D=off  SampleTime=-1
  Constant1 : Constant  Value=I_total
  Constant2 : Constant  Value=m_propellant
  Constant3 : Constant  Value=g
  Constant4 : Constant  Value=m_propellant
  Constant5 : Constant  Value=m_rocket
  Divide : Product  Inputs=*//
  Divide1 : Product  Inputs=*//
  Integrator : Integrator
  Product : Product
  Product1 : Product
  Scope : Scope
      settings: ActiveDisplayYMinimum=-0.10423  ActiveDisplayYMaximum=0.93803  DataLoggingVariableName=ScopeData2
  Scope5 : Scope
      settings: ActiveDisplayYMinimum=13.967875  ActiveDisplayYMaximum=16.859125
  m_dot : Outport
  m_roket : Outport  Port=2
  itki : Outport  Port=3
  wires:
  Add/1 -> Compare To Zero1/1, Product1/1
  Constant5/1 -> Add1/1
  1-D Lookup Table/1 -> Compare To Zero/1, Product/1  "İtki-zaman"
  Divide/1 -> m_dot/1, Scope/1, Integrator/1  "m_dot"
  Product1/1 -> Add1/2
  Constant4/1 -> Add/1
  Compare To Zero1/1 -> Product1/2
  Constant/1 -> Divide1/3
  Add1/1 -> m_roket/1, Scope5/1  "m_roket"
  Compare To Zero/1 -> Product/2
  Clock1/1 -> 1-D Lookup Table/1
  Integrator/1 -> Add/2
  Constant2/1 -> Divide1/2
  Product/1 -> Divide/1, itki/1
  Constant3/1 -> Divide/3
  Constant1/1 -> Divide1/1
  Divide1/1 -> Divide/2  "specific impulse"

== matlab function SonModel/MATLAB Function4 ==
  data: alpha_rad input; dCm_curve output; Mach input; dCm_table input; lut_valid output

function [dCm_curve, lut_valid] = DeltaCm_Curve_DI(alpha_rad, Mach, dCm_table)
%#codegen

% INPUTS:
% alpha_rad : AoA [rad]
% Mach      : Mach number
% dCm_table : 9x7x4 DeltaCm lookup table
%
% OUTPUTS:
% dCm_curve : 7x1 DeltaCm vector
% lut_valid : Validity of AoA and Mach

% Breakpoints
alpha_grid = [-10,-7.5,-5,-2.5,0,2.5,5,7.5,10] * pi/180;
mach_grid  = [0.20,0.40,0.70,0.84];

% Initialize outputs
dCm_curve = zeros(7,1);
lut_valid = false;

% Check AoA and Mach validity
if ~isfinite(alpha_rad) || ~isfinite(Mach)
    return;
end

% Check operating limits
if alpha_rad < alpha_grid(1) || ...
   alpha_rad > alpha_grid(9) || ...
   Mach < mach_grid(1) || ...
   Mach > mach_grid(4)

    % Outside KTS operating range
    % DeltaCm = 0
    return;
end

% Valid operating range
lut_valid = true;

a = alpha_rad;
m = Mach;

% Find AoA interval
ia = 8;

for i = 1:8
    if a <= alpha_grid(i+1)
        ia = i;
        break;
    end
end

% Find Mach interval
im = 3;

for k = 1:3
    if m <= mach_grid(k+1)
        im = k;
        break;
    end
end

% Interpolation weights
wa = (a-alpha_grid(ia)) / ...
     (alpha_grid(ia+1)-alpha_grid(ia));

wm = (m-mach_grid(im)) / ...
     (mach_grid(im+1)-mach_grid(im));

% Calculate DeltaCm for all 7 elevator angles
for j = 1:7

    c00 = dCm_table(ia,  j,im);
    c10 = dCm_table(ia+1,j,im);
    c01 = dCm_table(ia,  j,im+1);
    c11 = dCm_table(ia+1,j,im+1);

    % AoA interpolation
    lo = (1-wa)*c00 + wa*c10;
    hi = (1-wa)*c01 + wa*c11;

    % Mach interpolation
    dCm_curve(j) = (1-wm)*lo + wm*hi;

end

% Final validation
if ~all(isfinite(dCm_curve))
    dCm_curve = zeros(7,1);
    lut_valid = false;
end

end

== matlab function SonModel/MATLAB Function5 ==
  data: Xe input; x output; Ve input; x0 input; z_ground input; h output; gamma output; valid_motion output
function [x, h, gamma, valid_motion] = Flight_Signals(Xe, Ve, x0, z_ground)
%#codegen
% Xe, Ve: 3-element flat-Earth position [m] and GROUND velocity [m/s].
% x0: launch X coordinate. z_ground: target-ground downward coordinate.
% gamma is the projected X-h path angle, not a body or air-relative angle.
% Assumes negligible lateral motion and forward travel along Earth X.
x = Xe(1) - x0;
h = z_ground - Xe(3);
gamma = atan2(-Ve(3), Ve(1));
valid_motion = Ve(1) > 1.0; % numerical forward-motion guard, not a stall limit
end

== matlab function SonModel/MATLAB Function6 ==
  data: CN_mag input; CN_signed output; alpha_signed_rad input
function CN_signed = make_CN_signed(CN_mag, alpha_signed_rad)

if abs(alpha_signed_rad) < 1e-8
    CN_signed = 0;
else
    CN_signed = CN_mag * sign(alpha_signed_rad);
end

end

== matlab function SonModel/MATLAB Function7 ==
  data: F_raw input; F_applied output; M_raw input; X_e input; V_b input; X0_e input; M_applied output; on_rail output; s_rail output; rail_phase output; rail_clear_pulse output; rail_cleared_now output; V_exit_now output; F_rail_reaction output; M_rail_reaction output; rail_cleared_prev input; V_exit_prev input
function [F_applied, M_applied, on_rail, s_rail, ...
          rail_phase, rail_clear_pulse, ...
          rail_cleared_now, V_exit_now, ...
          F_rail_reaction, M_rail_reaction] = ...
          RailConstraint(F_raw, M_raw, X_e, V_b, ...
                                           X0_e, rail_cleared_prev, V_exit_prev)
%#codegen
%
% GOKTURK 1stageVson - IDEALIZED LAUNCH RAIL CONSTRAINT
% Geometry from supplied OpenRocket 23.09 .ork file (20 October 2026).
% Body axes: +X forward, +Y right, +Z down.
%
% VERIFIED FROM OPENROCKET:
%   Rocket length: 0.40 + 0.18 + 0.20 + 0.90 = 1.68 m
%   Rocket body diameter: 0.122 m
%   Physical launch rail: 6.00 m
%   Launch rod angle: 45 degrees from vertical (not applied here)
%   Launch altitude: 970 m (not applied here)
%
% ESTIMATED -- NOT PRESENT IN THE .ORK FILE:
%   Forward rail button: 0.72 m from nose
%       near forward fin root, spanning about 0.66-0.78 m
%   Aft rail button:     1.58 m from nose
%       near aft fin root, spanning about 1.48-1.68 m
%   REPLACE these with actual measured button positions before validation.
%
% All flags and rail_phase outputs are double for Simulink compatibility.
% Exit velocity is measured, not prescribed.

%% 1) GEOMETRY
L_rail   = 6.00;  % physical rail length [m] (OpenRocket)
L_rocket = 1.68;  % new rocket total length [m] (OpenRocket)

% ESTIMATES based on fin-root centers; no rail buttons defined in .ork.
x_button_front_nose = 0.72;  % [m] from nose; estimated
x_button_aft_nose   = 1.58;  % [m] from nose; estimated

x_button_front_tail = L_rocket - x_button_front_nose;  % 0.96 m
x_button_aft_tail   = L_rocket - x_button_aft_nose;    % 0.10 m

s_front_exit = L_rail - x_button_front_tail;  % 5.04 m
s_aft_exit   = L_rail - x_button_aft_tail;    % 5.90 m (complete release)

%% 2) DISTANCE TRAVELED SINCE INITIAL POSITION
% Model assumption: while guided, motion is strictly along the rail.
dX1 = X_e(1) - X0_e(1);
dX2 = X_e(2) - X0_e(2);
dX3 = X_e(3) - X0_e(3);
s_rail = sqrt(dX1*dX1 + dX2*dX2 + dX3*dX3);

%% 3) SPEED
u = V_b(1);
v = V_b(2);
w = V_b(3);
V_body = sqrt(u*u + v*v + w*w);

%% 4) CLEARANCE AND PERMANENT LATCH
was_cleared = rail_cleared_prev > 0.5;
clear_condition = s_rail >= s_aft_exit;

if was_cleared || clear_condition
    rail_cleared_now = 1.0;
else
    rail_cleared_now = 0.0;
end

%% 5) ONE-STEP EXIT PULSE
if (~was_cleared) && clear_condition
    rail_clear_pulse = 1.0;
else
    rail_clear_pulse = 0.0;
end

%% 6) RECORD ACTUAL EXIT SPEED
if rail_clear_pulse > 0.5
    V_exit_now = V_body;
else
    V_exit_now = V_exit_prev;
end

%% 7) RAIL PHASE
% 2: both buttons guided; 1: only aft button guided; 0: free.
if rail_cleared_now > 0.5
    rail_phase = 0.0;
elseif s_rail < s_front_exit
    rail_phase = 2.0;
else
    rail_phase = 1.0;
end

%% 8) APPLY IDEALIZED RAIL CONSTRAINT
if rail_cleared_now < 0.5
    on_rail = 1.0;
    Fx = F_raw(1);

    % Prevent backward axial acceleration at initial position.
    % Assumes F_raw(1) includes the axial component of gravity.
    position_tol = 1.0e-4;  % [m]
    velocity_tol = 1.0e-3;  % [m/s]
    if (s_rail <= position_tol) && ...
       (u <= velocity_tol) && ...
       (Fx < 0.0)
        Fx = 0.0;
    end

    % Allow the rail-aligned body X force only.
    F_applied = [Fx; 0.0; 0.0];

    % Rigid, idealized rail: cancel all applied moments until complete exit.
    M_applied = [0.0; 0.0; 0.0];

    % Reaction force/moment balance the constrained loads.
    F_rail_reaction = F_applied - F_raw;
    M_rail_reaction = M_applied - M_raw;
else
    on_rail = 0.0;
    F_applied = F_raw;
    M_applied = M_raw;
    F_rail_reaction = [0.0; 0.0; 0.0];
    M_rail_reaction = [0.0; 0.0; 0.0];
end
end

== matlab function SonModel/MATLAB Function8 ==
  data: CN0 input; Cm0 output; CG_m input; CP_m input; Lref input
function Cm0 = calc_Cm0(CN0, CG_m, CP_m, Lref)

% Base pitch moment coefficient
% CN0   : RASAero signed normal-force coefficient
% CG_m  : CG location from nose [m]
% CP_m  : CP location from nose [m]
% Lref  : reference length [m]

Cm0 = CN0 * (CG_m - CP_m) / Lref;

end

== matlab function SonModel/MATLAB Function9 ==
  data: Cm input; CN input; CA input; rho input; Sref input; Lref input; u input; F_aero_b output; w input; M_aero_b output
function [F_aero_b, M_aero_b] = aero_forces_moment_3DOF( ...
    Cm, CN, CA, rho, Sref, Lref, u, w)

% Body eksenleri:
% +X : ileri
% +Z : asagi
% +Y : pitch ekseni
%
% Cm : Cm0 + DeltaCm
% CN : CN0_signed + DeltaCN
% CA : CA0 + DeltaCA

%% Hava hizi
V = sqrt(u^2 + w^2);

if V < 1e-6
    F_aero_b = [0; 0; 0];
    M_aero_b = [0; 0; 0];
    return;
end

%% Dinamik basinc
qbar = 0.5 * rho * V^2;

%% Aerodinamik kuvvetler

% Axial kuvvet
% CA > 0 -> -X yonu
Fx = -qbar * Sref * CA;

% Normal kuvvet
% CN > 0 -> -Z yonu
Fz = -qbar * Sref * CN;

F_aero_b = [Fx;
            0;
            Fz];

%% Pitch momenti

My = qbar * Sref * Lref * Cm;

M_aero_b = [0;
            My;
            0];

end

== matlab function SonModel/MATLAB Function10 ==
  data: Mach input; Mach_LUT output; KTS_active output
function [Mach_LUT, KTS_active] = KTS_Mach_Control(Mach)

if Mach < 0.20
    Mach_LUT   = 0.20;
    KTS_active = 0;

elseif Mach > 0.84
    Mach_LUT   = 0.84;
    KTS_active = 1;

else
    Mach_LUT   = Mach;
    KTS_active = 1;
end

end
